simulink model "flightControlSystem"  (R2026b)
settings: Solver=ode3  StopTime=TFinal
PreLoadFcn:
  | InitVars;
  | definePX4ParamsBus;
undefined symbols (not defined in the file): control_power, DiscIntNeverNeededParam, init, MC_PITCHRATE_MAX, MC_ROLLRATE_MAX, MC_YAWRATE_MAX, PX4_Params_Default, SampleTime, timestamp
libraries: px4Utilslib x52, px4uORBlib x10, vrlib x8, aerolibutil x8, simulink x5, sharedutil x3, matrix_library x2, raspberrypiutilitieslib x2, px4Peripheralslib x2, sharedtransform x1, px4Sensorslib x1
(part 4 of 4)

== system flightControlSystem/MultiCopter Controller/Position & Altitude controller/Position controller/PositionVelocityControl/Position P control Loop/constrain ==
  vel_sp_z_raw_ms : Inport
  neg_MPC_Z_VEL_MAX_UP : Inport  Port=2
  MPC_Z_VEL_MAX_DN : Inport  Port=3
  Max : MinMax  Function=max  Inputs=2
  Min : MinMax  Inputs=2
  vel_sp_z_clamped_ms : Outport
  wires:
  vel_sp_z_raw_ms/1 -> Max/1
  neg_MPC_Z_VEL_MAX_UP/1 -> Max/2
  Max/1 -> Min/1
  MPC_Z_VEL_MAX_DN/1 -> Min/2
  Min/1 -> vel_sp_z_clamped_ms/1

== system flightControlSystem/MultiCopter Controller/Position & Altitude controller/Position controller/PositionVelocityControl/Position P control Loop/constrained_xy ==
  vel_sp_xy_2x1 : Inport
  vel_sp_feedfwd_xy_2x1 : Inport  Port=2
  MPC_XY_VEL_MAX_ms : Inport  Port=3
  Add : Sum
  Add1 : Sum
  Add2 : Sum
  Constant : Constant  Value=0.001  SampleTime=-1
  Constant1 : Constant  Value=0.001  SampleTime=-1
  Dot Product : DotProduct  OutDataTypeStr=Inherit: Inherit via internal rule
  Dot Product1 : DotProduct  OutDataTypeStr=Inherit: Inherit via internal rule
  Gain : Gain  Gain=-1
  Normalize Vector : vrlib/Utilities/Normalize Vector  maxzero=0
  Normalize Vector2 : vrlib/Utilities/Normalize Vector  maxzero=0
  Product1 : Product
  Product2 : Product
  Product3 : Product
  Relational Operator : RelationalOperator  Operator=<=  OutDataTypeStr=boolean  RndMeth=Simplest  InputSameDT=off
  Relational Operator1 : RelationalOperator  OutDataTypeStr=boolean  RndMeth=Simplest  InputSameDT=off
  Relational Operator2 : RelationalOperator  Operator=<  OutDataTypeStr=boolean  RndMeth=Simplest  InputSameDT=off
  Relational Operator3 : RelationalOperator  Operator=<  OutDataTypeStr=boolean  RndMeth=Simplest  InputSameDT=off
  Square : Math  Operator=square
  Square Root : Sqrt
  Square1 : Math  Operator=square
  Subtract : Sum  Inputs=+-
  Subtract1 : Sum  Inputs=+-
  Subtract2 : Sum  Inputs=+-
  Switch{,1..3} (4 alike) : Switch  Criteria=u2 > Threshold  SaturateOnIntegerOverflow=off  InputSameDT=off
  norm_vel_added_xy : MATLAB Function  TreatAsAtomicUnit=on
  norm_vel_feedfwd_xy : MATLAB Function  TreatAsAtomicUnit=on
  norm_vel_result_xy : MATLAB Function  TreatAsAtomicUnit=on
  norm_vel_sp_xy : MATLAB Function  TreatAsAtomicUnit=on
  vel_sp_xy_constrained_ms : Outport
  wires:
  Subtract/1 -> norm_vel_result_xy/1(u)
  vel_sp_xy_2x1/1 -> Add2/1, Dot Product1/1, Dot Product1/2, Dot Product/2, Add/1, norm_vel_added_xy/1(u), Subtract/2, Normalize Vector2/1, norm_vel_sp_xy/1(u)
  vel_sp_feedfwd_xy_2x1/1 -> Add/2, Subtract/1, Normalize Vector/1
  norm_vel_result_xy/1(y) -> Relational Operator2/1
  MPC_XY_VEL_MAX_ms/1 -> Square/1, Product3/2, Product2/2, Relational Operator/2, Relational Operator1/2
  Normalize Vector/1 -> Product1/1, Product3/1, Dot Product/1
  Product3/1 -> Switch3/1
  norm_vel_sp_xy/1(y) -> Relational Operator3/1
  Gain/1 -> Add1/1
  Normalize Vector2/1 -> Product2/1
  Constant1/1 -> Relational Operator3/2
  norm_vel_added_xy/1(y) -> Relational Operator1/1
  Relational Operator/1 -> Switch/2
  Add/1 -> Switch/1, norm_vel_feedfwd_xy/1(u)
  Square Root/1 -> Add1/2
  Dot Product/1 -> Gain/1, Square1/1
  Switch/1 -> Switch1/3
  Dot Product1/1 -> Subtract1/1
  Relational Operator2/1 -> Switch2/2
  Square/1 -> Subtract1/2
  Relational Operator3/1 -> Switch3/2
  Constant/1 -> Relational Operator2/2
  Relational Operator1/1 -> Switch1/2
  norm_vel_feedfwd_xy/1(y) -> Relational Operator/1
  Square1/1 -> Subtract2/1
  Subtract1/1 -> Subtract2/2
  Subtract2/1 -> Square Root/1
  Product2/1 -> Switch2/1, Switch1/1
  Add1/1 -> Product1/2
  Product1/1 -> Add2/2
  Add2/1 -> Switch/3
  Switch1/1 -> Switch2/3
  Switch3/1 -> vel_sp_xy_constrained_ms/1
  Switch2/1 -> Switch3/3

== system flightControlSystem/MultiCopter Controller/Position & Altitude controller/Position controller/PositionVelocityControl/acceleration_control/ACC_Decoupling ==
  thrust_body_previous_3x1 : Inport
  Constant : Constant  Value=9.81  OutDataTypeStr=double  SampleTime=-1
  DSR_MPC_ACC_DECOUPLE : DataStoreRead  DataStoreName=PX4_Params  DataStoreElements=PX4_Params.MPC_ACC_DECOUPLE  IndexOptions=Index vector (dialog)  Indices=1  OutputSizes=1
  Decouple_Switch : Switch  Threshold=1
  Sum_coupled : Sum  Inputs=+-
  tilt_correction_NED_ms2 : Outport
  wires:
  DSR_MPC_ACC_DECOUPLE/1 -> Decouple_Switch/2
  Sum_coupled/1 -> Decouple_Switch/3
  thrust_body_previous_3x1/1 -> Sum_coupled/2
  Decouple_Switch/1 -> tilt_correction_NED_ms2/1
  Constant/1 -> Sum_coupled/1, Decouple_Switch/1

== system flightControlSystem/MultiCopter Controller/Position & Altitude controller/Position controller/PositionVelocityControl/acceleration_control/limitTilt ==
  thrust_direction_body : Inport
  gravity_direction_NED : Inport  Port=2
  MPC_TILTMAX_AIR_rad : Inport  Port=3
  Acos : Trigonometry  Operator=acos
  Add : Sum
  Assignment : Assignment  DiagnosticForDimensions=Warning  IndexOptions=Index vector (dialog)  Indices=1  OutputSizes=1  RuntimeRangeChecks=off
  Constant : Constant  Value=eps('single');  SampleTime=-1
  Constant1 : Constant  SampleTime=-1
  Cos : Trigonometry  Operator=cos
  Divide : Product  Inputs=*/
  Dot Product : DotProduct  OutDataTypeStr=Inherit: Inherit via internal rule
  Dot Product1 : DotProduct  OutDataTypeStr=Inherit: Inherit via internal rule
  Min : MinMax  Inputs=2
  Product : Product
  Product1 : Product
  Product2 : Product
  Relational Operator : RelationalOperator  Operator=<  OutDataTypeStr=boolean  RndMeth=Simplest  InputSameDT=off
  Sin : Trigonometry
  Subtract : Sum  Inputs=+-
  Switch : Switch  Criteria=u2 > Threshold  SaturateOnIntegerOverflow=off  InputSameDT=off
  norm_thrust_vector : MATLAB Function  TreatAsAtomicUnit=on
  thrust_direction_tilt_limited : Outport
  wires:
  thrust_direction_body/1 -> Dot Product/1, Subtract/1
  gravity_direction_NED/1 -> Product/2, Product1/2, Dot Product/2
  Dot Product/1 -> Acos/1, Product/1
  Acos/1 -> Min/1
  MPC_TILTMAX_AIR_rad/1 -> Min/2
  Product/1 -> Subtract/2
  Constant/1 -> Relational Operator/2
  Subtract/1 -> Switch/3, Assignment/1, Dot Product1/1, Dot Product1/2
  Dot Product1/1 -> Relational Operator/1
  Relational Operator/1 -> Switch/2
  Constant1/1 -> Assignment/2
  Assignment/1 -> Switch/1
  Min/1 -> Sin/1, Cos/1
  Cos/1 -> Product1/1
  Sin/1 -> Product2/1
  norm_thrust_vector/1(y) -> Divide/2
  Switch/1 -> norm_thrust_vector/1(u), Divide/1
  Divide/1 -> Product2/2
  Product1/1 -> Add/1
  Product2/1 -> Add/2
  Add/1 -> thrust_direction_tilt_limited/1

== matlab function flightControlSystem/Actuator Commands/Simulation Actuator Commands/Mixer/MATLAB Function ==
  data: frameType input; rotor_cmd output size=[1 8]; thrust input; pitch input; roll input; yaw input
function rotor_cmd = MixerBlock(frameType, thrust, pitch, roll, yaw)
%#codegen
% Outputs a 1x8 vector for bus conversion

    rotor_cmd = zeros(1,8); % Always 8 motors

    % Select mixer matrix
    if frameType == "Quad+"
        mixer = [1,0,-1,1;
                 1,0,1,1;
                 1,1,0,-1;
                 1,-1,0,-1];
        N = 4;
    elseif frameType == "QuadX"
        mixer = [1,1,-1,1;
                 1,-1,1,1;
                 1,-1,-1,-1;
                 1,1,1,-1];
        N = 4;
    elseif frameType == "QuadH"
        mixer = [1,1,-1,1;
                 1,-1,1,1;
                 1,-1,-1,-1;
                 1,1,1,-1]; % Yaw    (from rotorDir)

        N = 4;
	elseif frameType == "Hexa+"
		s60 = sqrt(3)/2;
		c60 = 1/2;
		mixer = [
			1,  1,  0,  -1;           
			1, -1,  0,  1;           
			1, -0.5, -s60,  -1;            
			1,  0.5,  s60,  1;            
			1,  0.5, -s60,  1;            
			1, -0.5,  s60,  -1];           
		N = 6;
	elseif frameType == "HexaX"
		mixer = [
			1,  0,  1, -1;   
			1,  0, -1,  1;  
			1,  1, -1, -1;   
			1, -1,  1,  1;   
			1,  1,  1,  1;  
			1, -1, -1, -1    
			];
		N = 6;
    % elseif frameType == "OctoX"
    %     mixer = [1, 1, 0, 1;
    %              1, 0, -1, 1;
    %              1, -1, 0, 1;
    %              1, 0, 1, 1;
    %              1, 1, 0, -1;
    %              1, 0, -1, -1;
    %              1, -1, 0, -1;
    %              1, 0, 1, -1];
    %     N = 8;
    else
        mixer = zeros(4,4);
        N = 4;
    end

    ctrl = [thrust; pitch; roll; yaw];
    rotor = mixer * ctrl;
    rotor_cmd(1:N) = reshape(rotor,1,[]);
end

== matlab function flightControlSystem/MultiCopter Controller/Attitude_Controller/AttitudeControl/DCM_Z_FromQuat_Error ==
  data: q input; v output
function v = dcmZ(q)
    % Corresponding body z-axis to an attitude quaternion
    a = q(1);
    b = q(2);
    c = q(3);
    d = q(4);
    v = [2 * (a * c + b * d);
         2 * (c * d - a * b);
         a * a - b * b - c * c + d * d];
end

== matlab function flightControlSystem/MultiCopter Controller/Attitude_Controller/AttitudeControl/Canonical_Quaternion ==
  data: q input; q_canonical output
function q_canonical = canonical(q)
    % Return canonical form of the quaternion
    % Iterate over quaternion elements to find the first non-negligible component
    % and use its sign to adjust the quaternion to its canonical form.

    epsilon = eps('single'); % Equivalent to FLT_EPSILON in C++
    
    for i = 1:4
        if abs(q(i)) > epsilon
            q_canonical = q * single(sign(q(i)));
            return;
        end
    end

    % If all components are negligible (unlikely for a valid quaternion),
    % return the original quaternion.
    q_canonical = single(q);
end

== matlab function flightControlSystem/MultiCopter Controller/Attitude_Controller/AttitudeControl/Canonical_Quaternion_2 ==
  data: q input; q_canonical output
function q_canonical = canonical(q)
    % Return canonical form of the quaternion
    % Iterate over quaternion elements to find the first non-negligible component
    % and use its sign to adjust the quaternion to its canonical form.

    epsilon = eps('single'); % Equivalent to FLT_EPSILON in C++
    
    for i = 1:4
        if abs(q(i)) > epsilon
            q_canonical = q * single(sign(q(i)));
            return;
        end
    end

    % If all components are negligible (unlikely for a valid quaternion),
    % return the original quaternion.
    q_canonical = single(q);
end

== matlab function flightControlSystem/MultiCopter Controller/Attitude_Controller/AttitudeControl/DCM_Z_FromQuat_Desired ==
  data: q input; v output
function v = dcmZ(q)
    % Corresponding body z-axis to an attitude quaternion
    a = q(1);
    b = q(2);
    c = q(3);
    d = q(4);
    v = [2 * (a * c + b * d);
         2 * (c * d - a * b);
         a * a - b * b - c * c + d * d];
end

== matlab function flightControlSystem/MultiCopter Controller/Attitude_Controller/AttitudeControl/QuatImaginary_ToRateSetpoint ==
  data: q input; v output
function v = quatImag(q)
    % Imaginary part of quaternion
    v = q(2:4);
end

== matlab function flightControlSystem/MultiCopter Controller/Angular Rate Control/ControlPower_Monitor ==
  data: vehicle_torque_setpoint input; dt input; control_power output
function control_power = updateActuatorControlsStatus(vehicle_torque_setpoint, dt)
	persistent control_energy energy_integration_time
	
	if isempty(control_energy)
		control_energy = zeros(1, 3);
		energy_integration_time = 0;
	end
	
	control_power = zeros(1, 3);
	
	% Update control energy
	for i = 1:3
		control_energy(i) = control_energy(i) + vehicle_torque_setpoint(i) * vehicle_torque_setpoint(i) * dt;
	end
	
	% Update energy integration time
	energy_integration_time = energy_integration_time + dt;
	
	% Check if integration time exceeds threshold
	if energy_integration_time > 500e-3
	
		for i = 1:3
			control_power(i) = control_energy(i) / energy_integration_time;
			control_energy(i) = 0;
		end

		% Reset integration time
		energy_integration_time = 0;
	end
end

== matlab function flightControlSystem/MultiCopter Controller/Angular Rate Control/RatePID_Core/YawTorqueLPF_v116 ==
  data: yaw_torque input; yaw_torque_filt output; dt input; MC_YAW_TQ_CUTOFF input
function yaw_torque_filt = YawTorqueLPF_v116(yaw_torque, dt, MC_YAW_TQ_CUTOFF)
%#codegen
% PX4 v1.16 yaw torque low-pass filter
% Insertion point: after rate controller PID, before actuator mixer
% Reference: MulticopterRateControl.cpp
%   torque_setpoint(2) = _output_lpf_yaw.update(torque_setpoint(2), dt)
%
% Uses same AlphaFilter formula as velocity LP:
%   b = 2*pi*fc*dt; a = b/(1+b); state = a*input + (1-a)*state

persistent yaw_lp_state initialized

if isempty(initialized)
    yaw_lp_state = 0;
    initialized = true;
end

% AlphaFilter::update(sample, dt)
b = 2*pi*MC_YAW_TQ_CUTOFF*dt;
a = b / (1 + b);
yaw_lp_state = a * yaw_torque + (1 - a) * yaw_lp_state;
yaw_torque_filt = yaw_lp_state;

== matlab function flightControlSystem/MultiCopter Controller/Position & Altitude controller/Position controller/PositionVelocityControl/Position P control Loop/VelSP_Combine_PosError/addIfNotNan_VelSP_Plus_Feedfwd ==
  data: setpoint input; setpoint output; addition input
function setpoint = addIfNotNanVector3f(setpoint, addition)
    for i = 1:3
        setpoint(i) = addIfNotNan(setpoint(i), addition(i));
    end
end

function value = addIfNotNan(value, addition)
    value = single(value);
    if isfinite(value) && isfinite(addition)
        value = value + addition;
    elseif ~isfinite(value)
        value = single(addition);
    end
    % If addition is NaN or both are NaN, do nothing
end

== matlab function flightControlSystem/MultiCopter Controller/Attitude_Controller/EulerToQuaternion_Setpoint ==
  data: roll input; qd output; pitch input; yaw input
function qd = eulerToQuaternion(roll, pitch, yaw)
    % Convert roll, pitch, yaw (in radians) to a quaternion
    cr = cos(roll / 2);
    sr = sin(roll / 2);
    cp = cos(pitch / 2);
    sp = sin(pitch / 2);
    cy = cos(yaw / 2);
    sy = sin(yaw / 2);

    qd = [cr * cp * cy + sr * sp * sy, ...
          sr * cp * cy - cr * sp * sy, ...
          cr * sp * cy + sr * cp * sy, ...
          cr * cp * sy - sr * sp * cy];
	qd = qd / norm(qd);
end

== matlab function flightControlSystem/Actuator Commands/Actuator Commands/MATLAB Function ==
  data: y output
function y = fcn()

y =  zeros(1,8);

== matlab function flightControlSystem/SetpointManager/Set target Position/Landing Logic/PX4 Landing Logic ==
  data: land_trigger input; pos_sp output; states input; MPC_LAND_SPEED_in input; MPC_LAND_CRWL_in input; MPC_LAND_ALT1_in input; MPC_LAND_ALT2_in input; MPC_LAND_ALT3_in input; MPC_Z_VEL_MAX_DN_in input; vel_sp output; acc_sp output
function [pos_sp, vel_sp, acc_sp] = PX4LandingLogic(land_trigger, states, MPC_LAND_SPEED_in, MPC_LAND_CRWL_in, MPC_LAND_ALT1_in, MPC_LAND_ALT2_in, MPC_LAND_ALT3_in, MPC_Z_VEL_MAX_DN_in)
%#codegen
% PX4 v1.16.2 style multi-phase landing logic
% states = [X, Y, Z, Yaw] from getcurrentState bus
% In this controller: POSITIVE Vz = DESCEND (more thrust reduction)

persistent X_lock Y_lock Yaw_lock triggered
if isempty(triggered)
    triggered = false;
    X_lock = 0;
    Y_lock = 0;
    Yaw_lock = 0;
end

% Capture X, Y, Yaw on rising edge of land_trigger
if land_trigger > 0 && ~triggered
    X_lock = states(1);
    Y_lock = states(2);
    Yaw_lock = states(4);
    triggered = true;
elseif land_trigger == 0
    triggered = false;
end

if land_trigger > 0
    % Compute altitude above ground (positive up)
    altitude = -states(3);  % NED: Z negative = above ground

    % Multi-phase descent speed (PX4 v1.16.2)
    if altitude > MPC_LAND_ALT1_in
        land_speed = MPC_Z_VEL_MAX_DN_in;
    elseif altitude > MPC_LAND_ALT2_in
        frac = (altitude - MPC_LAND_ALT2_in) / (MPC_LAND_ALT1_in - MPC_LAND_ALT2_in);
        land_speed = MPC_LAND_SPEED_in + frac * (MPC_Z_VEL_MAX_DN_in - MPC_LAND_SPEED_in);
    elseif altitude > MPC_LAND_ALT3_in
        land_speed = MPC_LAND_SPEED_in;
    else
        land_speed = MPC_LAND_CRWL_in;
    end

    % Position: lock X,Y; NaN for Z (velocity-controlled); lock Yaw
    pos_sp = [X_lock, Y_lock, nan, Yaw_lock];

    % Velocity: zero XY, positive Vz for descent
    vel_sp = [0, 0, land_speed];

    % Acceleration: zero (no feedforward)
    acc_sp = [0, 0, 0];
else
    pos_sp = [0, 0, 0, 0];
    vel_sp = [0, 0, 0];
    acc_sp = [0, 0, 0];
end
end

== matlab function flightControlSystem/MultiCopter Controller/Position & Altitude controller/Position controller/PositionVelocityControl/Position P control Loop/VelSP_Combine_PosError/setZeroIfNan_VelSP ==
  data: vector input; vector output
function vector = setZeroIfNanVector3f(vector)
    vector = addIfNotNanVector3f(vector, [0; 0; 0]);
end

% Function to add if not NaN for a 3-element vector
function setpoint = addIfNotNanVector3f(setpoint, addition)
for i = 1:3
    setpoint(i) = addIfNotNan(setpoint(i), addition(i));
end
end

% Function to add if not NaN
function value = addIfNotNan(value, addition)
value = single(value);
if isfinite(value) && isfinite(addition)
    value = value + addition;
elseif ~isfinite(value)
    value = single(addition);
end
% If addition is NaN or both are NaN, do nothing
end

== matlab function flightControlSystem/MultiCopter Controller/Position & Altitude controller/Position controller/PositionVelocityControl/Position P control Loop/constrained_xy/norm_vel_sp_xy ==
  data: u input; y output
function y = fcn(u)

y = norm(u);

== matlab function flightControlSystem/MultiCopter Controller/Position & Altitude controller/Position controller/PositionVelocityControl/Position P control Loop/constrained_xy/norm_vel_added_xy ==
  data: u input; y output
function y = fcn(u)

y = norm(u);

== matlab function flightControlSystem/MultiCopter Controller/Position & Altitude controller/Position controller/PositionVelocityControl/Position P control Loop/constrained_xy/norm_vel_feedfwd_xy ==
  data: u input; y output
function y = fcn(u)

y = norm(u);

== matlab function flightControlSystem/MultiCopter Controller/Position & Altitude controller/Position controller/PositionVelocityControl/thrust_allocation/setZeroIfNan_ThrustSP ==
  data: vector input; vector output
function vector = setZeroIfNanVector3f(vector)
    vector = addIfNotNanVector3f(vector, [0; 0; 0]);
end

% Function to add if not NaN for a 3-element vector
function setpoint = addIfNotNanVector3f(setpoint, addition)
for i = 1:3
    setpoint(i) = addIfNotNan(setpoint(i), addition(i));
end
end

% Function to add if not NaN
function value = addIfNotNan(value, addition)
value = single(value);
if isfinite(value) && isfinite(addition)
    value = value + addition;
elseif ~isfinite(value)
    value = single(addition);
end
% If addition is NaN or both are NaN, do nothing
end

== matlab function flightControlSystem/SetpointManager/Simulation Set target Position/Landing Logic/PX4 Landing Logic ==
  data: land_trigger input; pos_sp output; states input; MPC_LAND_SPEED_in input; MPC_LAND_CRWL_in input; MPC_LAND_ALT1_in input; MPC_LAND_ALT2_in input; MPC_LAND_ALT3_in input; MPC_Z_VEL_MAX_DN_in input; vel_sp output; acc_sp output
function [pos_sp, vel_sp, acc_sp] = PX4LandingLogic(land_trigger, states, MPC_LAND_SPEED_in, MPC_LAND_CRWL_in, MPC_LAND_ALT1_in, MPC_LAND_ALT2_in, MPC_LAND_ALT3_in, MPC_Z_VEL_MAX_DN_in)
%#codegen
% PX4 v1.16.2 style multi-phase landing logic
% states = [X, Y, Z, Yaw] from getcurrentState bus
% In this controller: POSITIVE Vz = DESCEND (more thrust reduction)

persistent X_lock Y_lock Yaw_lock triggered
if isempty(triggered)
    triggered = false;
    X_lock = 0;
    Y_lock = 0;
    Yaw_lock = 0;
end

% Capture X, Y, Yaw on rising edge of land_trigger
if land_trigger > 0 && ~triggered
    X_lock = states(1);
    Y_lock = states(2);
    Yaw_lock = states(4);
    triggered = true;
elseif land_trigger == 0
    triggered = false;
end

if land_trigger > 0
    % Compute altitude above ground (positive up)
    altitude = -states(3);  % NED: Z negative = above ground

    % Multi-phase descent speed (PX4 v1.16.2)
    if altitude > MPC_LAND_ALT1_in
        land_speed = MPC_Z_VEL_MAX_DN_in;
    elseif altitude > MPC_LAND_ALT2_in
        frac = (altitude - MPC_LAND_ALT2_in) / (MPC_LAND_ALT1_in - MPC_LAND_ALT2_in);
        land_speed = MPC_LAND_SPEED_in + frac * (MPC_Z_VEL_MAX_DN_in - MPC_LAND_SPEED_in);
    elseif altitude > MPC_LAND_ALT3_in
        land_speed = MPC_LAND_SPEED_in;
    else
        land_speed = MPC_LAND_CRWL_in;
    end

    % Position: lock X,Y; NaN for Z (velocity-controlled); lock Yaw
    pos_sp = [X_lock, Y_lock, nan, Yaw_lock];

    % Velocity: zero XY, positive Vz for descent
    vel_sp = [0, 0, land_speed];

    % Acceleration: zero (no feedforward)
    acc_sp = [0, 0, 0];
else
    pos_sp = [0, 0, 0, 0];
    vel_sp = [0, 0, 0];
    acc_sp = [0, 0, 0];
end
end

== matlab function flightControlSystem/Estimator/Estimator/DeltaTime_PositionCtrl ==
  data: timestamp_sample input; dt output
function dt = calculateDeltaTime(timestamp_sample)

    persistent time_stamp_last_loop;

    % Initialize _time_stamp_last_loop if it's empty
    if isempty(time_stamp_last_loop)
        time_stamp_last_loop = hrt_absolute_time();
    end

    % Calculate dt with constraints
    dt = constrain(((timestamp_sample - time_stamp_last_loop) * 1e-6), 0.002, 0.04);

    % Update _time_stamp_last_loop for the next iteration
    time_stamp_last_loop = timestamp_sample;
end

function value = constrain(value, min_val, max_val)
    % Constrain the value between min_val and max_val
    value = max(min(value, max_val), min_val);
end

function abs_time_us = hrt_absolute_time()
    % Initialize a persistent variable to store the start time
    persistent start_time;
    
    % If this is the first call, set the start time using tic
    if isempty(start_time)
        start_time = tic;
    end
    
    % Get the elapsed time since the start in seconds
    elapsed_time_sec = toc(start_time);
    
    % Convert elapsed time to microseconds
    abs_time_us = elapsed_time_sec * 1e6;
end

== matlab function flightControlSystem/MultiCopter Controller/Position & Altitude controller/Position controller/PositionVelocityControl/Position P control Loop/constrained_xy/norm_vel_result_xy ==
  data: u input; y output
function y = fcn(u)

y = norm(u);

== matlab function flightControlSystem/MultiCopter Controller/Position & Altitude controller/Position controller/PositionVelocityControl/IgnoreOpticalFlow_till_25cm/TakeoffRamp_VelZ_Limiter ==
  data: vel_sp_z input; vel_sp_z_limited output; dt input
function vel_sp_z_limited = TakeoffRamp(vel_sp_z, dt)
%#codegen
%TakeoffRamp  PX4 v1.16 takeoff velocity ramp
%  This LIMITS the maximum upward velocity - it does NOT override the
%  position controller. The position controller still controls to target
%  altitude; this just prevents it from commanding too much climb rate
%  during the first few seconds (which causes thrust transient → drift).
%
%  vel_sp_z comes FROM the position P-controller (already computed from
%  altitude error). This block only clamps it, never makes it climb faster.

persistent state elapsed ramp_progress

COM_SPOOLUP_TIME = 1.0;   % Motor spool-up (seconds)
MPC_TKO_RAMP_T  = 3.0;    % Ramp duration (seconds)
MPC_TKO_SPEED   = 1.5;    % Max takeoff climb rate (m/s, positive up)
MPC_Z_VEL_P     = 4.0;    % Z velocity P-gain (your Constant8(3))

if isempty(state)
    state = uint8(0);       % 0=spoolup, 1=rampup, 2=flight
    elapsed = 0.0;
    ramp_progress = 0.0;
end

% Zero-thrust velocity: vel_sp that makes velocity PID output ≈ 0
ramp_vz_init = -9.81 / max(MPC_Z_VEL_P, 0.01);  % ≈ -2.45 m/s (NED)

switch state
    case uint8(0)
        % SPOOLUP: clamp to zero-thrust velocity (motors spinning up)
        % Position controller may want to climb, but we don't allow it yet
        vel_sp_z_limited = max(vel_sp_z, ramp_vz_init);
        elapsed = elapsed + dt;
        if elapsed >= COM_SPOOLUP_TIME
            state = uint8(1);
        end

    case uint8(1)
        % RAMPUP: gradually open the velocity limit
        if MPC_TKO_RAMP_T > 0
            ramp_progress = min(ramp_progress + dt / MPC_TKO_RAMP_T, 1.0);
        else
            ramp_progress = 1.0;
        end

        % Current velocity ceiling (interpolate from ramp_vz_init to -TKO_SPEED)
        vel_limit = ramp_vz_init + ramp_progress * (-MPC_TKO_SPEED - ramp_vz_init);

        % CLAMP: position controller's vel_sp cannot exceed this limit
        % In NED: more negative = faster climb. max() picks the slower (less negative).
        % If pos controller wants -0.5 m/s and limit is -1.0 → pass -0.5 (within limit)
        % If pos controller wants -3.0 m/s and limit is -1.0 → clamp to -1.0
        vel_sp_z_limited = max(vel_sp_z, vel_limit);

        if ramp_progress >= 1.0
            state = uint8(2);
        end

    case uint8(2)
        % FLIGHT: no limiting, position controller has full authority
        vel_sp_z_limited = vel_sp_z;

    otherwise
        vel_sp_z_limited = vel_sp_z;
end
end

== matlab function flightControlSystem/MultiCopter Controller/Position & Altitude controller/Position controller/PositionVelocityControl/Hover_Thrust/HoverThrustEKF_ZeroOrder ==
  data: az input; hover_thrust_estimate output; thrust input; dt input; vx input; vy input; vz input; mpc_hover_thrust input
function hover_thrust_estimate = hoverThrustEstimator(az, thrust, dt, vx, vy, vz, mpc_hover_thrust)
    % Constants
    CONSTANTS_ONE_G = single(9.81); % Gravity constant

    acc_z = az;
    % Persistent variables to maintain state across function calls
    persistent hover_thr hover_thr_min hover_thr_max gate_size state_var process_var acc_var acc_var_scale
    persistent innov innov_var innov_test_ratio residual_lpf signed_innov_test_ratio_lpf
    persistent noise_learning_time_constant lpf_time_constant valid param_updated

    mpc_thr_hover = mpc_hover_thrust;
    hte_thr_range = single(0.2);
    hte_vz_thr = single(2);
    hte_vxy_thr = single(10);
    hte_ht_noise = single(0.0036);
    hte_ht_err_init = single(0.1);
    hte_acc_gate = single(3);
    in_air = single(1);
    armed = single(1);

    if isempty(hover_thr)
        % Initialize parameters
        hover_thr = single(0.5);
        hover_thr_min = single(0.1);
        hover_thr_max = single(0.9);
        gate_size = single(3.0);
        state_var = single(0.01);
        process_var = single(12.5e-6);
        acc_var = single(5.0);
        acc_var_scale = single(1.0);
        innov = single(0.0);
        innov_var = single(0.0);
        innov_test_ratio = single(0.0);
        residual_lpf = single(0.0);
        signed_innov_test_ratio_lpf = single(0.0);
        noise_learning_time_constant = single(2.0);
        lpf_time_constant = single(1.0);
        valid = false;
    end

    % Update parameters if needed
    if isempty(param_updated)
        hover_thr_min = single(max(mpc_thr_hover - hte_thr_range, 0.0));
        hover_thr_max = single(min(mpc_thr_hover + hte_thr_range, 1.0));
        process_var = hte_ht_noise^2;
        state_var = hte_ht_err_init^2;
        gate_size = hte_acc_gate;
        param_updated = true;
    end

    % Check preconditions
    if armed && in_air && (dt > 0.001) && (dt < 1.0) && isfinite(az)
        % Predict step
        state_var = state_var + process_var * dt^2;

        % Calculate measurement noise coefficients
        meas_noise_coeff_z = max((abs(vz) - hte_vz_thr) + 1.0, 1.0);
        meas_noise_coeff_xy = max(norm_v([vx, vy]) - hte_vxy_thr + 1.0, 1.0);
        acc_var_scale = max(meas_noise_coeff_xy, meas_noise_coeff_z);

        % Measurement update
        H = -CONSTANTS_ONE_G * thrust / hover_thr^2;
        innov_var = max(H * state_var * H + acc_var * acc_var_scale, acc_var * acc_var_scale);
        predicted_acc_z = CONSTANTS_ONE_G * thrust / hover_thr - CONSTANTS_ONE_G;
        innov = acc_z - predicted_acc_z;
        K = state_var * H / innov_var;
        innov_test_ratio = innov^2 / (gate_size^2 * innov_var);

        % Update state if innovation test passes
        if innov_test_ratio < 1
            hover_thr = max(min(hover_thr + K * innov, hover_thr_max), hover_thr_min);
            state_var = max((1 - K * H) * state_var, 1e-10);
        elseif abs(signed_innov_test_ratio_lpf) > 0.2
            state_var = state_var + 1e3 * process_var * dt^2;
        end

        % Update low-pass filters
        alpha = dt / (lpf_time_constant + dt);
        residual = innov;
        residual_lpf = (1 - alpha) * residual_lpf + alpha * residual;
        signed_innov_test_ratio_lpf = (1 - alpha) * signed_innov_test_ratio_lpf + alpha * sign(innov) * innov_test_ratio;

        % Update measurement noise
        alpha = dt / (noise_learning_time_constant + dt);
        res_no_bias = residual - residual_lpf;
        acc_var = max((1 - alpha) * acc_var + alpha * (res_no_bias^2 + H * state_var * H), 1);

        % Update valid state
        if valid
            valid = valid && innov_test_ratio < 1;
        else
            valid = innov_test_ratio < 1 && state_var < 0.001;
        end
    end

    % Output the estimated hover thrust
    hover_thrust_estimate = hover_thr;
end

function v = norm_squared(v)
v = dot_v(v,v);
end

function v = length_v(v)
v = norm_v(v);
end

function v = norm_v(v)
v = sqrt(dot_v(v,v));
end

function v = unit_v(v)
v = v/norm_v(v);
end

function v = normalised_v(v)
v = unit_v(v);
end

function r = dot_v(a, b)
% a is a vector (1D array)
% b is a matrix
% The function computes the dot product of vector a with the first column of matrix b

% Ensure a is a column vector
a = a(:);

% Initialize the result
r = single(0);

% Get the number of elements in the vector
M = length(a);

% Compute the dot product with the first column of b
for i = 1:M
    r = r + a(i) * b(i);
end
end

== matlab function flightControlSystem/MultiCopter Controller/Position & Altitude controller/Position controller/PositionVelocityControl/thrust_allocation/norm_thrust_xy_magnitude ==
  data: u input; y output
function y = fcn(u)

y = norm(u);

== matlab function flightControlSystem/SetpointManager/Set target Position/RC Failsafe Signal/MATLAB Function ==
  data: status input; out output; ch7 input; RSSI input
function out = rcLatch(status, ch7, RSSI)
%#codegen
% Inputs:
%   status - scalar (e.g., uint8 or double)
%   ch7    - scalar (e.g., uint16 or double)
%   RSSI   - scalar (e.g., uint8 or double)
% Output:
%   out    - scalar (0 or 1)

persistent prevOut
if isempty(prevOut)
    prevOut = 0;
end

if status == 0 && RSSI ~= 0
    if ch7 > 1600
        prevOut = 1;
    elseif ch7 < 1600
        prevOut = 0;
    end
end

out = prevOut;
end

== matlab function flightControlSystem/MultiCopter Controller/Position & Altitude controller/Position controller/PositionVelocityControl/Velocity_Control/addIfNotNan_AccSP_Feedfwd ==
  data: setpoint input; setpoint output; addition input
% Function to add if not NaN for a 3-element vector
function setpoint = addIfNotNanVector3f(setpoint, addition)
    for i = 1:3
        setpoint(i) = addIfNotNan(setpoint(i), addition(i));
    end
end

% Function to add if not NaN
function value = addIfNotNan(value, addition)
	value = single(value);
    if isfinite(value) && isfinite(addition)
        value = value + addition;
    elseif ~isfinite(value)
        value = single(addition);
    end
    % If addition is NaN or both are NaN, do nothing
end

== matlab function flightControlSystem/MultiCopter Controller/Position & Altitude controller/Position controller/PositionVelocityControl/acceleration_control/limitTilt/norm_thrust_vector ==
  data: u input; y output
function y = fcn(u)

y = norm(u);

== matlab function flightControlSystem/MultiCopter Controller/Position & Altitude controller/Position controller/thrustToAttitude/RotMat_To_Euler_RPY ==
  data: body_x input; y output; body_y input; body_z input
function y = fcn(body_x, body_y, body_z)

y = rotm2eul([body_x, body_y, body_z],'ZYX');

== matlab function flightControlSystem/Estimator/Estimator/DeltaTime_AttitudeCtrl ==
  data: timestamp_sample input; dt output
function dt = calculateDeltaTime(timestamp_sample)

    persistent time_stamp_last_loop;

    % Initialize _time_stamp_last_loop if it's empty
    if isempty(time_stamp_last_loop)
        time_stamp_last_loop = hrt_absolute_time();
    end

    % Calculate dt with constraints
    dt = constrain(((timestamp_sample - time_stamp_last_loop) * 1e-6), 0.002, 0.02);

    % Update _time_stamp_last_loop for the next iteration
    time_stamp_last_loop = timestamp_sample;
end

function value = constrain(value, min_val, max_val)
    % Constrain the value between min_val and max_val
    value = max(min(value, max_val), min_val);
end

function abs_time_us = hrt_absolute_time()
    % Initialize a persistent variable to store the start time
    persistent start_time;
    
    % If this is the first call, set the start time using tic
    if isempty(start_time)
        start_time = tic;
    end
    
    % Get the elapsed time since the start in seconds
    elapsed_time_sec = toc(start_time);
    
    % Convert elapsed time to microseconds
    abs_time_us = elapsed_time_sec * 1e6;
end

== matlab function flightControlSystem/MultiCopter Controller/Position & Altitude controller/Position controller/TiltLimit_SlewRate ==
  data: dt input; tilt_limit_deg input; lim_tilt output
function lim_tilt = updateSlewRateYaw(dt, tilt_limit_deg)
    % Define persistent variables to hold state across function calls
    persistent value slewrate
    
    % Initialize persistent variables on the first call
    if isempty(value)
        value = 0; % Initial value
    end
    if isempty(slewrate)
        slewrate = 0.2; % Slew rate
    end
    
    % Convert tilt limit from degrees to radians
    tilt_limit_rad = deg2rad(tilt_limit_deg);
    new_value = tilt_limit_rad;
    % Update slewrate with yaw wrapping [-pi, pi]
    d_wrapped = wrap_pi(new_value - value);
    updated_value = wrap_pi(updateSlewRate(value + d_wrapped, dt));
    
    % Update the persistent value
    value = updated_value;
    
    % Assign the updated value to lim_tilt
    lim_tilt = value;
end

function updated_value = updateSlewRate(new_value, dt)
    % Define persistent variables for the SlewRate function
    persistent value slewrate
    
    % Initialize persistent variables on the first call
    if isempty(value)
        value = 0; % Initial value
    end
    if isempty(slewrate)
        slewrate = 0.2; % Slew rate
    end
    
    % Limit the rate of change of the value
    dvalue_desired = new_value - value;
    dvalue_max = slewrate * dt;
    dvalue = constrain(dvalue_desired, -dvalue_max, dvalue_max);
    
    % Update the persistent value
    value = value + dvalue;
    updated_value = value;
end

function result = constrain(value, min_val, max_val)
    % Constrain value between min_val and max_val
    result = min(max(value, min_val), max_val);
end

function wrapped_angle = wrap_pi(angle)
    % Wrap the angle to the range [-π, π)

    % Define the low and high bounds
    low = -pi;
    high = pi;

    % Calculate the range
    range = high - low;

    % Check if the angle is already within the desired range
    if low <= angle && angle < high
        wrapped_angle = angle;
        return;
    end

    % Calculate the number of wraps and adjust the angle
    num_wraps = floor((angle - low) / range);
    wrapped_angle = angle - range * num_wraps;
end

== matlab function flightControlSystem/MultiCopter Controller/Position & Altitude controller/Position controller/thrustToAttitude/ThrustMagnitude_Norm ==
  data: u input; y output
function y = fcn(u)

y = norm(u);

== matlab function flightControlSystem/Estimator/Estimator/DeltaTime_RateCtrl ==
  data: timestamp_sample input; dt output
function dt = calculateDeltaTime(timestamp_sample)

    persistent time_stamp_last_loop;

    % Initialize _time_stamp_last_loop if it's empty
    if isempty(time_stamp_last_loop)
        time_stamp_last_loop = hrt_absolute_time();
    end

    % Calculate dt with constraints
    dt = constrain(((timestamp_sample - time_stamp_last_loop) * 1e-6), 0.002, 0.04);

    % Update _time_stamp_last_loop for the next iteration
    time_stamp_last_loop = timestamp_sample;
end

function value = constrain(value, min_val, max_val)
    % Constrain the value between min_val and max_val
    value = max(min(value, max_val), min_val);
end

function abs_time_us = hrt_absolute_time()
    % Initialize a persistent variable to store the start time
    persistent start_time;
    
    % If this is the first call, set the start time using tic
    if isempty(start_time)
        start_time = tic;
    end
    
    % Get the elapsed time since the start in seconds
    elapsed_time_sec = toc(start_time);
    
    % Convert elapsed time to microseconds
    abs_time_us = elapsed_time_sec * 1e6;
end

== matlab function flightControlSystem/Estimator/Simulation Estimator/DeltaTime_Compute ==
  settings: updateMethod=DISCRETE
  data: u input; dt output
function dt = compute_dt(u)
%#codegen
persistent t_prev
if isempty(t_prev)
    t_prev = 0;
end

t_now = u;
dt = t_now - t_prev;
t_prev = t_now;

== matlab function flightControlSystem/MultiCopter Controller/Attitude_Controller/AttitudeControl/DCM_Z_FromQuat_Current ==
  data: q input; v output
function v = dcmZ(q)
    % Corresponding body z-axis to an attitude quaternion
    a = q(1);
    b = q(2);
    c = q(3);
    d = q(4);
    v = [2 * (a * c + b * d);
         2 * (c * d - a * b);
         a * a - b * b - c * c + d * d];
end

== matlab function flightControlSystem/Estimator/Simulation Estimator/ControlAllocator_Feedback ==
  data: control_setpoint input; unallocated_torque output; torque_setpoint_achieved output
function [unallocated_torque, torque_setpoint_achieved] = ctrl_allocator(control_setpoint)

control_allocation_scale =([1,1,1]);
effectiveness = ([1,1,1]);
actuator_sp = ([0,0,0]);
actuator_trim = ([0,0,0]);
allocated_control = (effectiveness .* (actuator_sp - actuator_trim)) .* control_allocation_scale;
unallocated_control = control_setpoint - allocated_control;

unallocated_torque = unallocated_control(1:3);
torque_setpoint_achieved = norm(unallocated_torque)^2 < 1e-6;
end

== matlab function flightControlSystem/MultiCopter Controller/Attitude_Controller/AttitudeControl/vectorToQuaternion/MATLAB Function ==
  data: src input; q output; dst input
function q = quatFromVectors(src, dst)
    % Quaternion from two vectors using single precision
    eps = single(1e-5);
    
    src = single(src(:)); % Ensure column vector and single precision
    dst = single(dst(:)); % Ensure column vector and single precision

    cr = cross(src, dst);
    dt = dot(src, dst);

	if norm(cr) < eps && dt < 0
		% Handle 180 degree rotation
		cr = abs(src);
		if cr(1) < cr(2)
			if cr(1) < cr(3)
				cr = single([1; 0; 0]);
			else
				cr = single([0; 0; 1]);
			end
		else
			if cr(2) < cr(3)
				cr = single([0; 1; 0]);
			else
				cr = single([0; 0; 1]);
			end
		end
		q0 = single(0);
		cr = cross(src, cr);
	else
		% Normal case, do half-way quaternion solution
		q0 = dt + sqrt(dot(src,src) * dot(dst,dst));
	end

    q = single([q0; cr(1); cr(2); cr(3)]);
end

== matlab function flightControlSystem/Estimator/Simulation Estimator/EulerToQuat_SetpointConversion ==
  data: roll input; qd output; pitch input; yaw input
function qd = eulerToQuaternion(roll, pitch, yaw)
    % Convert roll, pitch, yaw (in radians) to a quaternion
    cr = cos(roll / 2);
    sr = sin(roll / 2);
    cp = cos(pitch / 2);
    sp = sin(pitch / 2);
    cy = cos(yaw / 2);
    sy = sin(yaw / 2);

    qd = [cr * cp * cy + sr * sp * sy, ...
          sr * cp * cy - cr * sp * sy, ...
          cr * sp * cy + sr * cp * sy, ...
          cr * cp * sy - sr * sp * cy];
	qd = qd / norm(qd);
end

== matlab function flightControlSystem/Estimator/Simulation Estimator/QDelta_BetweenSteps ==
  data: q_curr input; q_Delta output; q_prev input
function q_Delta = computeDeltaQuaternion(q_curr, q_prev)
% computeDeltaQuaternion - Computes the delta quaternion between two orientations
%
% Syntax: q_Delta = computeDeltaQuaternion(q_curr, q_prev)
%
% Inputs:
%   q_curr - current quaternion (1x4 vector or quaternion object)
%   q_prev - previous quaternion (1x4 vector or quaternion object)
%
% Output:
%   q_Delta - delta quaternion (1x4 vector)

% Ensure inputs are row vectors
q_curr = reshape(q_curr, 1, []);
q_prev = reshape(q_prev, 1, []);

% Compute the delta quaternion
q_Delta = quatmultiply(q_curr, quatinv(q_prev));

% Normalize the result
q_Delta = q_Delta / norm(q_Delta);
end

== matlab function flightControlSystem/Estimator/Estimator/set_vehicle_states_v116 ==
  data: x input; position output; y input; z input; vx input; vy input; vz input; heading input; xy_valid input; z_valid input; v_xy_valid input; v_z_valid input; dt input; MPC_VEL_NF_FRQ input; MPC_VEL_NF_BW input; MPC_VEL_LP input; MPC_VELD_LP input; velocity output; acceleration output; yaw output
function [position, velocity, acceleration, yaw] = set_vehicle_states_v116(x, y, z, vx, vy, vz, heading, xy_valid, z_valid, v_xy_valid, v_z_valid, dt, MPC_VEL_NF_FRQ, MPC_VEL_NF_BW, MPC_VEL_LP, MPC_VELD_LP)
%#codegen
% PX4 v1.16 set_vehicle_states — drop-in replacement for MATLAB Function5
% Reference: PX4-Autopilot/src/modules/mc_pos_control/MulticopterPositionControl.cpp
%
% v1.16 changes vs v1.14:
%   1. Velocity notch filter (removes frame vibration at MPC_VEL_NF_FRQ)
%   2. Velocity low-pass filter (MPC_VEL_LP Hz, smooths before D-term)
%   3. Derivative computed on LP-filtered signal (getState - prev_state)/dt
%   4. Derivative LP filter (MPC_VELD_LP Hz, same as v1.14 cutoff)
%
% AlphaFilter formula: tau=1/(2*pi*fc); alpha=dt/(dt+tau)
%   which equals: b=2*pi*fc*dt; a=b/(1+b) — same as v1.14 BlockLowPass

persistent notch_x1_xy notch_x2_xy notch_y1_xy notch_y2_xy
persistent notch_x1_z notch_x2_z notch_y1_z notch_y2_z
persistent vel_lp_state_xy vel_lp_state_z
persistent deriv_lp_state_x deriv_lp_state_y deriv_lp_state_z
persistent initialized

if isempty(initialized)
    notch_x1_xy = zeros(2,1); notch_x2_xy = zeros(2,1);
    notch_y1_xy = zeros(2,1); notch_y2_xy = zeros(2,1);
    notch_x1_z = 0; notch_x2_z = 0;
    notch_y1_z = 0; notch_y2_z = 0;
    vel_lp_state_xy = zeros(2,1);
    vel_lp_state_z = 0;
    deriv_lp_state_x = 0;
    deriv_lp_state_y = 0;
    deriv_lp_state_z = 0;
    initialized = true;
end

% Outputs
position = [x, y, z];
velocity = [vx, vy, vz];
acceleration = [0, 0, 0];
yaw = heading;

sample_freq = 1/dt;

% --- Notch filter coefficients (computed once, same for XY and Z) ---
if MPC_VEL_NF_FRQ > 0 && MPC_VEL_NF_BW > 0 && MPC_VEL_NF_FRQ < sample_freq/2
    alpha_n = tan(pi * MPC_VEL_NF_BW / sample_freq);
    beta_n = -cos(2*pi * MPC_VEL_NF_FRQ / sample_freq);
    a0_inv = 1 / (alpha_n + 1);
    b0 = a0_inv; b1_n = 2*beta_n*a0_inv; b2 = a0_inv;
    a1_n = b1_n; a2_n = (1 - alpha_n)*a0_inv;
    notch_enabled = true;
else
    b0=1; b1_n=0; b2=0; a1_n=0; a2_n=0;
    notch_enabled = false;
end

% --- LP filter alpha (velocity) ---
if MPC_VEL_LP > 0
    b_lp = 2*pi*MPC_VEL_LP*dt;
    alpha_lp = b_lp / (1 + b_lp);
    lp_enabled = true;
else
    alpha_lp = 1;
    lp_enabled = false;
end

% --- LP filter alpha (derivative) ---
b_d = 2*pi*MPC_VELD_LP*dt;
alpha_d = b_d / (1 + b_d);

% ============================================
% XY VELOCITY PROCESSING
% ============================================
velocity_xy = [vx; vy];

% Stage 1: Notch filter (PX4 NotchFilter::apply, Direct Form I)
if notch_enabled
    vel_notched_xy = b0*velocity_xy + b1_n*notch_x1_xy + b2*notch_x2_xy ...
                     - a1_n*notch_y1_xy - a2_n*notch_y2_xy;
    notch_x2_xy = notch_x1_xy; notch_x1_xy = velocity_xy;
    notch_y2_xy = notch_y1_xy; notch_y1_xy = vel_notched_xy;
else
    vel_notched_xy = velocity_xy;
end

% Stage 2: Velocity LP (PX4 AlphaFilter::update)
% _vel_xy_lp_filter.getState() — save BEFORE update
vel_xy_prev = vel_lp_state_xy;

if lp_enabled
    % state = state + alpha * (sample - state)
    vel_lp_state_xy = vel_lp_state_xy + alpha_lp * (vel_notched_xy - vel_lp_state_xy);
else
    vel_lp_state_xy = vel_notched_xy;
end

% states.velocity.xy() = _vel_xy_lp_filter.update(...)
velocity(1:2) = vel_lp_state_xy;

% Stage 3: Derivative LP (PX4 FilteredDerivative via AlphaFilter)
% deriv = (_vel_xy_lp_filter.getState() - vel_xy_prev) / dt_s
deriv_xy = (vel_lp_state_xy - vel_xy_prev) / dt;

% _vel_deriv_xy_lp_filter.update(deriv)
deriv_lp_state_x = deriv_lp_state_x + alpha_d * (deriv_xy(1) - deriv_lp_state_x);
deriv_lp_state_y = deriv_lp_state_y + alpha_d * (deriv_xy(2) - deriv_lp_state_y);
acceleration(1) = deriv_lp_state_x;
acceleration(2) = deriv_lp_state_y;

% ============================================
% Z VELOCITY PROCESSING
% ============================================

% Stage 1: Notch filter Z
if notch_enabled
    vel_notched_z = b0*vz + b1_n*notch_x1_z + b2*notch_x2_z ...
                    - a1_n*notch_y1_z - a2_n*notch_y2_z;
    notch_x2_z = notch_x1_z; notch_x1_z = vz;
    notch_y2_z = notch_y1_z; notch_y1_z = vel_notched_z;
else
    vel_notched_z = vz;
end

% Stage 2: Velocity LP Z
vel_z_prev = vel_lp_state_z;
if lp_enabled
    vel_lp_state_z = vel_lp_state_z + alpha_lp * (vel_notched_z - vel_lp_state_z);
else
    vel_lp_state_z = vel_notched_z;
end
velocity(3) = vel_lp_state_z;

% Stage 3: Derivative LP Z
deriv_z = (vel_lp_state_z - vel_z_prev) / dt;
deriv_lp_state_z = deriv_lp_state_z + alpha_d * (deriv_z - deriv_lp_state_z);
acceleration(3) = deriv_lp_state_z;
